simulink model "Hydroelectric Power Model"  (R2026a)
settings: Solver=VariableStepAuto  StopTime=0.1
StartFcn:
  | learning.simulink.modelCallbacks.startFunction(gcs);
StopFcn:
  | learning.simulink.modelCallbacks.stopFunction(gcs);learning.assess.assessments.student.StudentBlockValue.updateForSimulation(gcs);
model workspace (MAT data in the model file):
  courseObject.course = 'simscape'
  courseObject.chapter = 6
  courseObject.lesson = 4
  courseObject.section = 1
  courseObject.task = 1
undefined symbols (not defined in the file): b, Dh, g, h_res, K_gen, r_load, rho
libraries: fl_lib x17, nesl_utility x1
CloseFcn:
  | learning.simulink.cleanupOnlineTraining;learning.simulink.Application.getInstance().dduxLogMatlabEvent("ModelClosed");
Description:
  | TrainingCourseModel
settings Model: SimulationMode=accelerator  Creator=PC  LastModifiedBy=PC
settings SimscapeCC: SimscapeNominalValues="[{\"value\":\"1\",\"unit\":\"A\"},{\"value\":\"1\",\"unit\":\"bar\"},{\"value\":\"1\",\"unit\":\"cm^2\"},{\"value\":\"1\",\"unit\":\"cm^3/s\"},{\"value\":\"1\",\"unit\":\"kJ/kg\"},{\"value\":\"1\",\"unit\":\"kW\"},{\"value\":\"1\",\"unit\":\"l\"},{\"value\":\"1\",\"unit\":\"N\"},{\"value\":\"1\",\"unit\":\"N*m\"},{\"value\":\"1\",\"unit\":\"V\"}]"  SimscapeLogLimitData=off  SimscapeLogDataHistory=5000.0

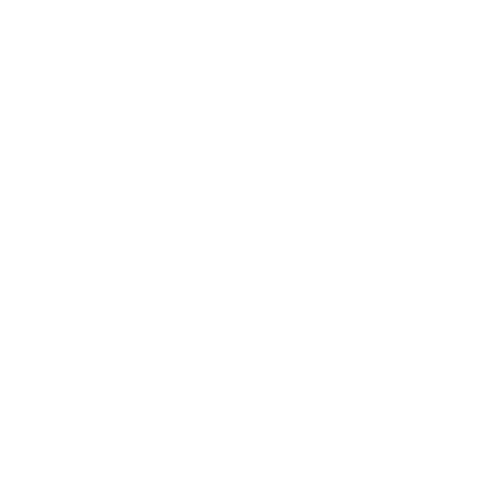
[thumbnail: Simulink's stored preview of the top-level diagram]
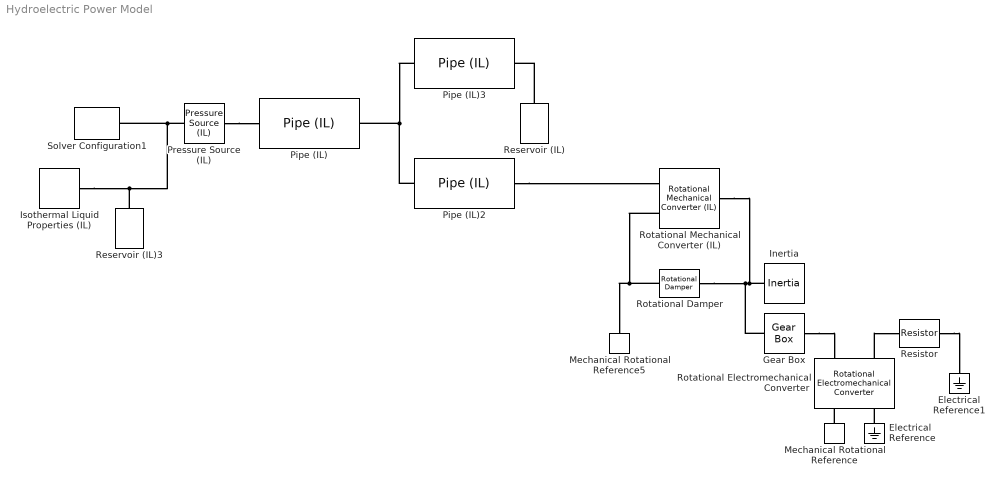
== system Hydroelectric Power Model ==
  Electrical Reference : fl_lib/Electrical/Electrical Elements/Electrical Reference
  Electrical Reference1 : fl_lib/Electrical/Electrical Elements/Electrical Reference
  Gear Box : fl_lib/Mechanical/Mechanisms/Gear Box  ratio=R_gear  t_in_specify=off  t_in_priority=None  t_in=0 N*m  t_in_nominal_specify=off  t_in_nominal_value=1  t_in_nominal_unit=N*m  t_out_specify=off  t_out_priority=None  t_out=0 N*m  t_out_nominal_specify=off  t_out_nominal_value=1  t_out_nominal_unit=N*m
  Inertia : fl_lib/Mechanical/Rotational Elements/Inertia  inertia=I_wheel kg*m^2  num_ports=foundation.enum.numPorts2.one  w_specify=off  w_priority=High  w=0 rad/s  w_nominal_specify=off  w_nominal_value=1  w_nominal_unit=rad/s  t_specify=off  t_priority=None  t=0 N*m  t_nominal_specify=off  t_nominal_value=1  t_nominal_unit=N*m
  Isothermal Liquid Properties (IL) : fl_lib/Isothermal Liquid/Utilities/Isothermal Liquid Properties (IL)  rho_L_atm=998.21 kg/m^3  bulk_modulus_model=foundation.enum.bulk_modulus_model.const  beta_gain=6  beta_L_atm=2.1791e9 Pa  nu_atm=1.0034e-6 m^2/s  p_atm=0.101325 MPa  p_min=0.1 Pa  properties_range_check=simscape.enum.assert.action.error  air_fraction=0  polytropic_index=1.0  rho_g_atm=1.225 kg/m^3  air_dissolution_model=simscape.enum.onoff.off  p_crit=3 MPa
  Mechanical Rotational Reference : fl_lib/Mechanical/Rotational Elements/Mechanical Rotational Reference
  Mechanical Rotational Reference5 : fl_lib/Mechanical/Rotational Elements/Mechanical Rotational Reference
  Pipe (IL) : fl_lib/Isothermal Liquid/Elements/Pipe (IL)  length=pipe_length m  area=pi*(Dh/2)^2 m^2  Dh=Dh m  length_add=1 m  roughness=15e-6 m  Re_lam=2000  Re_tur=4000  shape_factor=64  dynamic_compressibility=simscape.enum.onoff.on  inertia=simscape.enum.onoff.off  p0=0.101325 MPa  mdot0=0 kg/s
  Pipe (IL)2 : fl_lib/Isothermal Liquid/Elements/Pipe (IL)  length=pipe_length m  area=pi*(Dh/2)^2 m^2  Dh=Dh m  length_add=1 m  roughness=15e-6 m  Re_lam=2000  Re_tur=4000  shape_factor=64  dynamic_compressibility=simscape.enum.onoff.on  inertia=simscape.enum.onoff.off  p0=0.101325 MPa  mdot0=0 kg/s
  Pipe (IL)3 : fl_lib/Isothermal Liquid/Elements/Pipe (IL)  length=pipe_length m  area=pi*(Dh/2)^2 m^2  Dh=Dh m  length_add=1 m  roughness=15e-6 m  Re_lam=2000  Re_tur=4000  shape_factor=64  dynamic_compressibility=simscape.enum.onoff.on  inertia=simscape.enum.onoff.off  p0=0.101325 MPa  mdot0=0 kg/s
  Pressure Source (IL) : fl_lib/Isothermal Liquid/Sources/Pressure Source (IL)  source_type=foundation.enum.constant_controlled.constant  pressure_differential=rho*g*h_res Pa
  Reservoir (IL) : fl_lib/Isothermal Liquid/Elements/Reservoir (IL)  pressure_input=false  pressure_spec=foundation.enum.pressure_spec.atmospheric  reservoir_pressure=0.101325 MPa
  Reservoir (IL)3 : fl_lib/Isothermal Liquid/Elements/Reservoir (IL)  pressure_input=false  pressure_spec=foundation.enum.pressure_spec.atmospheric  reservoir_pressure=0.101325 MPa
  Resistor : fl_lib/Electrical/Electrical Elements/Resistor  R=r_load Ohm  i_specify=off  i_priority=None  i=0 A  i_nominal_specify=off  i_nominal_value=1  i_nominal_unit=A  v_specify=off  v_priority=None  v=0 V  v_nominal_specify=off  v_nominal_value=1  v_nominal_unit=V
  Rotational Electromechanical Converter : fl_lib/Electrical/Electrical Elements/Rotational Electromechanical Converter  K=K_gen V/(rad/s)  i_specify=off  i_priority=None  i=0 A  i_nominal_specify=off  i_nominal_value=1  i_nominal_unit=A  v_specify=off  v_priority=None  v=0 V  v_nominal_specify=off  v_nominal_value=1  v_nominal_unit=V  t_specify=off  t_priority=None  t=0 N*m  t_nominal_specify=off  t_nominal_value=1  t_nominal_unit=N*m  w_specify=off  w_priority=None  w=0 rad/s  w_nominal_specify=off  w_nominal_value=1  w_nominal_unit=rad/s
  Rotational Mechanical Converter (IL) : fl_lib/Isothermal Liquid/Elements/Rotational Mechanical Converter (IL)  mech_orientation=foundation.enum.MechOrientationRotational.Positive  rotation_spec=foundation.enum.RotationSpec.Calculate  theta0=0 rad  volume_displacement=vol_displacement m^3/rad  dead_volume=1e-5 m^3  pressure_spec=foundation.enum.pressure_spec.atmospheric  environment_pressure=0.101325 MPa  dynamic_compressibility=true  p0=0.101325 MPa  p_nominal=0.101325 MPa
  Rotational Damper : fl_lib/Mechanical/Rotational Elements/Rotational Damper  D=b N*m/(rad/s)  w_specify=off  w_priority=None  w=0 rad/s  w_nominal_specify=off  w_nominal_value=1  w_nominal_unit=rad/s  t_specify=off  t_priority=None  t=0 N*m  t_nominal_specify=off  t_nominal_value=1  t_nominal_unit=N*m
  Solver Configuration1 : nesl_utility/Solver Configuration  PhysicalDomain=network_engine_domain  SubClassName=solver  LeftPortType=input  RightPortType=generic  Tones=[]  Harmonics=[]  SimulateNoise=off  Profile=off  UseLocalSampling=off  EnableSwitchedLinearOptims=on  FrequencyDomain=off  UseCCode=off  RelTol=0.001  AbsTol=1e-06  MinStep=1e-09  ToWorkspace=off  RevertToSquareIcSolve=off  NumHomotopyIterations=100  PhasorMode=off  PhasorModeNumHarmonics=1  ConsistencySolver=NEWTON_FTOL  CanonicalOrdering=UNORDERED  OptimizeIntermediates=UNOPTIMIZED  IndexReductionMethod=DerivativeReplacement  DoDC=off  ResidualTolerance=1e-09  ConsistencyTolSource=GLOBAL  ConsistencyAbsTol=0.001  ConsistencyRelTol=0.001  ConsistencyTolFactor=0.001  UseLocalSolver=off  LocalSolverChoice=NE_BACKWARD_EULER_ADVANCER  ResolveIndetEquations=on  FunctionEvalNumThread=1  LocalSolverSampleTime=0.001  DoFixedCost=off  MaxNonlinIter=3  MaxModeIter=2  ComputeImpulses=off  ImpulseIterations=1  LinearAlgebra=auto  LinearAlgebraNumThread=0  EquationFormulation=NE_TIME_EF  DelaysMemoryBudget=1024  AutomaticFiltering=on  FilteringTimeConstant=0.001  PartitionStorageMethod=AS_NEEDED  PartitionMemoryBudget=1024  PartitionMethod=ROBUST  MultibodyUseLocalSolver=off  MultibodyLocalSolverChoice=ODE1  MultibodyLocalSolverSampleTime=0.001
  connections:
  Solver Configuration1/RConn1 -- Pressure Source (IL)/LConn1 -- Isothermal Liquid Properties (IL)/RConn1 -- Reservoir (IL)3/LConn1
  Rotational Damper/RConn1 -- Rotational Mechanical Converter (IL)/RConn1 -- Inertia/LConn1 -- Gear Box/LConn1
  Pipe (IL)/RConn1 -- Pipe (IL)2/LConn1 -- Pipe (IL)3/LConn1
  Rotational Damper/LConn1 -- Rotational Mechanical Converter (IL)/LConn2 -- Mechanical Rotational Reference5/LConn1
  Gear Box/RConn1 -- Rotational Electromechanical Converter/LConn2
  Mechanical Rotational Reference/LConn1 -- Rotational Electromechanical Converter/RConn2
  Pipe (IL)2/RConn1 -- Rotational Mechanical Converter (IL)/LConn1
  Rotational Electromechanical Converter/LConn1 -- Resistor/LConn1
  Reservoir (IL)/LConn1 -- Pipe (IL)3/RConn1
  Pressure Source (IL)/RConn1 -- Pipe (IL)/LConn1
  Resistor/RConn1 -- Electrical Reference1/LConn1
  Electrical Reference/LConn1 -- Rotational Electromechanical Converter/RConn1
